simulink model "BandPassFilterSystem"  (R2023b)
settings: Solver=VariableStepAuto  StartTime=0.0  StopTime=5e-3  RelTol=1e-3
libraries: simulink x1
settings Model: Creator=rlschie  LastModifiedBy=rlschie

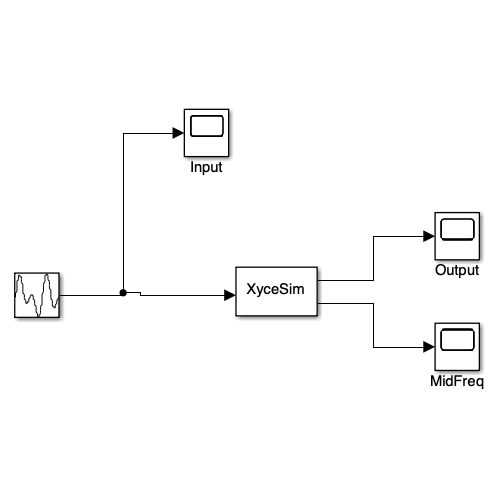
[thumbnail: Simulink's stored preview of the top-level diagram]
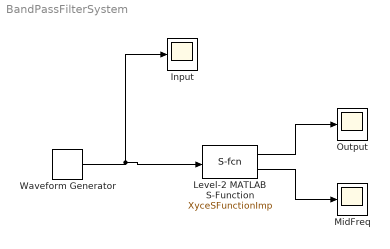
== system BandPassFilterSystem ==
  Input : Scope
  Level-2 MATLAB S-Function : M-S-Function  FunctionName=XyceSFunctionImp  Parameters=XyceInputFileName,WorkingDirectory,NumberOfInputs,NumberOfOutputs,InputNames,OutputNames  mask{XyceInputFileName=BandPassFilter.cir, WorkingDirectory=/Users/rlschie/src/XyceDevelopment/Xyce/utils/SimulinkInterface/SimulinkExamples/, XyceInputPortNames=, XyceOutputPortNames=, XyceNumberOfInputPorts=0, XyceNumberOfOutputPorts=0, NumberOfInputs=1, NumberOfOutputs=2, InputNames={ '1', 'YDAC!DAC_DRIVER' }, OutputNames={ '1', 'YADC!ADC_OUT'; '2', 'YADC!ADC_MID' }}
      mask prompts: XyceInputFileName "Xyce Input Filename"; WorkingDirectory "Working Directory"; XyceInputPortNames "Xyce Input Port Names"; XyceOutputPortNames "Xyce Output Port Names"; XyceNumberOfInputPorts "Xyce Number Of Inputs"; XyceNumberOfOutputPorts "Xyce Number Of Outputs"; NumberOfInputs "Number of Inputs"; NumberOfOutputs "Number of Outputs"; InputNames "Input Names"; OutputNames "Output Names"
      mask DialogControl SelectXyceInputFileButton Prompt: Select Xyce Input File
      mask DialogControl ScanXyceInputFileButton Prompt: Scan Xyce Input File
      mask DialogControl ResetForm Prompt: Reset
      mask DialogControl AddInputLineButton Prompt: Add Line
      mask DialogControl RemoveInputLineButton Prompt: Remove Line
      mask DialogControl AddOutputLineButton Prompt: Add Line
      mask DialogControl RemoveOutputLineButton Prompt: Remove Line
      mask Display: disp('XyceSim');
  MidFreq : Scope
  Output : Scope
  Waveform Generator : simulink/Sources/Waveform Generator  OutMin=[]  OutMax=[]  OutDataTypeStr=double  SelectedSignal=1  Signals=sin('Amplitude', 5, 'Frequency', 2*pi*100) + sin('Amplitude',2, 'Frequency',2*pi*2000, 'Phase', pi) + sin('Amplitude',1, 'Frequency',2*pi*20000,'Phase',0.25*pi)  BlockNames=MultiportSwitch_d8f2aab784cb4a9  SampleTime=1e-5
  wires:
  Waveform Generator/1 -> Level-2 MATLAB S-Function/1, Input/1
  Level-2 MATLAB S-Function/1 -> Output/1
  Level-2 MATLAB S-Function/2 -> MidFreq/1
